simulink model "GFMUPS100k_CPP"  (R2024b)
settings: Solver=ode2  StartTime=0.0  StopTime=6  FixedStep=5e-7  RelTol=1e-3
model workspace (MAT data in the model file):
  amp = 0
  f1 = 1000
undefined symbols (not defined in the file or in its folder): DiscIntNeverNeededParam, L
libraries: spsIGBTDiodeLib x12, slpidlib x12, spsabctodq0Lib x10, spsSeriesRLCBranchLib x9, spsPLL3phLib x8, spsThreePhaseSeriesRLCBranchLib x8, spsDiodeLib x6, dspstat3 x5, spsVoltageMeasurementLib x4, spsThreePhaseVIMeasurementLib x4, spsPower3phInstantaneousLib x3, spsControlledCurrentSourceLib x3
(part 2 of 4)

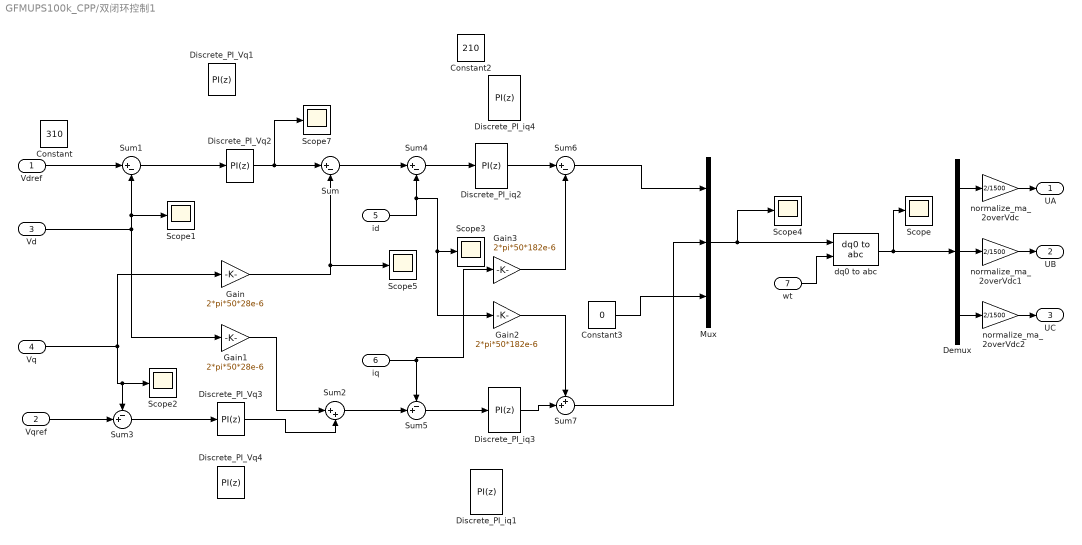
== system GFMUPS100k_CPP/双闭环控制1 ==
  Vdref : Inport
  Vqref : Inport  Port=2
  Vd : Inport  Port=3
  Vq : Inport  Port=4
  id : Inport  Port=5
  iq : Inport  Port=6
  wt : Inport  Port=7
  Constant : Constant  Value=310
  Constant2 : Constant  Value=210
  Constant3 : Constant  Value=0
  Demux : Demux  Outputs=3
  Discrete_PI_Vq1 : slpidlib/PID Controller  Controller=PI  Form=Parallel  TimeDomain=Discrete-time  UseExternalTs=off  SampleTime=5e-05  IntegratorMethod=Forward Euler  FilterMethod=Forward Euler  ControllerParametersSource=internal  P=0.16  I=500  UseKiTs=off  D=0  UseExternalDerivativeSource=off  N=100  UseFilter=on  TunerSelectOption=Transfer Function Based (PID Tuner App)  InitialConditionSource=internal  InitialConditionForIntegrator=0  InitialConditionForFilter=0  DifferentiatorICPrevScaledInput=0  ExternalReset=none  TrackingMode=off  Kt=1  LimitOutput=off  SatLimitsSource=internal  UpperSaturationLimit=inf  LowerSaturationLimit=-inf  LinearizeAsGain=off  AntiWindupMode=none  Kb=1  LimitIntegrator=off  UpperIntegratorSaturationLimit=inf  LowerIntegratorSaturationLimit=-inf  POutMin=[]  POutMax=[]  IOutMin=[]  IOutMax=[]  DOutMin=[]  DOutMax=[]  NOutMin=[]  NOutMax=[]  SumOutMin=[]  SumOutMax=[]  SaturationOutMin=[]  SaturationOutMax=[]  PParamMin=[]  PParamMax=[]  IParamMin=[]  IParamMax=[]  DParamMin=[]  DParamMax=[]  NParamMin=[]  NParamMax=[]  KbParamMin=[]  KbParamMax=[]  KtParamMin=[]  KtParamMax=[]  KbOutMin=[]  KbOutMax=[]  KtOutMin=[]  KtOutMax=[]  IntegratorOutMin=[]  IntegratorOutMax=[]  FilterOutMin=[]  FilterOutMax=[]  SumI1OutMin=[]  SumI1OutMax=[]  SumI2OutMin=[]  SumI2OutMax=[]  SumI3OutMin=[]  SumI3OutMax=[]  SumI4OutMin=[]  SumI4OutMax=[]  SumDOutMin=[]  SumDOutMax=[]  DifferentiatorOutMin=[]  DifferentiatorOutMax=[]  FilterDiffOutCoefMin=[]  FilterDiffOutCoefMax=[]  ReciprocalOutMin=[]  ReciprocalOutMax=[]  SumDenOutMin=[]  SumDenOutMax=[]  SumNumOutMin=[]  SumNumOutMax=[]  DivideOutMin=[]  DivideOutMax=[]  UdiffTsProdOutMin=[]  UdiffTsProdOutMax=[]  NTsProdOutMin=[]  NTsProdOutMax=[]  UintegralTsProdOutMin=[]  UintegralTsProdOutMax=[]  UngainTsProdOutMin=[]  UngainTsProdOutMax=[]  ClampingZeroOutDataTypeStr=Inherit: Inherit via back propagation  ClampingZeroOutMin=[]  ClampingZeroOutMax=[]  FilterDenConstantOutDataTypeStr=Inherit: Inherit via back propagation  FilterDenConstantOutMin=[]  FilterDenConstantOutMax=[]  PCopyOutDataTypeStr=Inherit: Inherit via back propagation  PCopyOutMin=[]  PCopyOutMax=[]  NCopyOutDataTypeStr=Inherit: Inherit via back propagation  NCopyOutMin=[]  NCopyOutMax=[]  IntegratorContinuousStateAttributes=''  IntegratorStateMustResolveToSignalObject=off  IntegratorRTWStateStorageClass=Auto  FilterContinuousStateAttributes=''  FilterStateMustResolveToSignalObject=off  FilterRTWStateStorageClass=Auto  ParallelPVariant=InternalParameters  IdealPVariant=Disabled  IVariant=InternalParameters  DVariant=Disabled  IntegratorVariant=Discrete  SatVariant=Disabled  AWVariant=Passthrough  PCopyVariant=Disabled  TRVariant=Disabled  FdbkBlocksVariant=Forward  IdealPFdbkVariant=Disabled  SatFdbkVariant=Disabled  DerivativeFilterVariant=Disabled  NVariant=Disabled  NCopyVariant=Disabled_SignalSpec  FilterICVariant=Disabled  IntegratorICVariant=InternalICs  ExternalResetVariant=Disabled  TRSumVariant=Passthrough  SumFdbkVariant=Disabled  SumVariant=Sum_PI  TsampFilterVariant=InternalTs  TsampNgainVariant=Passthrough  TsampIntegralVariant=Disabled_SignalSpec  ExternalSaturationOutDataTypeStr=Inherit: Same as second input  DerivativeSourceVariant=Disabled  PreIntVariant=InternalPreInt
  Discrete_PI_Vq2 : slpidlib/PID Controller  Controller=PI  Form=Parallel  TimeDomain=Discrete-time  UseExternalTs=off  SampleTime=5e-05  IntegratorMethod=Forward Euler  FilterMethod=Forward Euler  ControllerParametersSource=internal  P=0.16  I=250  UseKiTs=off  D=0  UseExternalDerivativeSource=off  N=100  UseFilter=on  TunerSelectOption=Transfer Function Based (PID Tuner App)  InitialConditionSource=internal  InitialConditionForIntegrator=0  InitialConditionForFilter=0  DifferentiatorICPrevScaledInput=0  ExternalReset=none  TrackingMode=off  Kt=1  LimitOutput=off  SatLimitsSource=internal  UpperSaturationLimit=inf  LowerSaturationLimit=-inf  LinearizeAsGain=off  AntiWindupMode=none  Kb=1  LimitIntegrator=off  UpperIntegratorSaturationLimit=inf  LowerIntegratorSaturationLimit=-inf  POutMin=[]  POutMax=[]  IOutMin=[]  IOutMax=[]  DOutMin=[]  DOutMax=[]  NOutMin=[]  NOutMax=[]  SumOutMin=[]  SumOutMax=[]  SaturationOutMin=[]  SaturationOutMax=[]  PParamMin=[]  PParamMax=[]  IParamMin=[]  IParamMax=[]  DParamMin=[]  DParamMax=[]  NParamMin=[]  NParamMax=[]  KbParamMin=[]  KbParamMax=[]  KtParamMin=[]  KtParamMax=[]  KbOutMin=[]  KbOutMax=[]  KtOutMin=[]  KtOutMax=[]  IntegratorOutMin=[]  IntegratorOutMax=[]  FilterOutMin=[]  FilterOutMax=[]  SumI1OutMin=[]  SumI1OutMax=[]  SumI2OutMin=[]  SumI2OutMax=[]  SumI3OutMin=[]  SumI3OutMax=[]  SumI4OutMin=[]  SumI4OutMax=[]  SumDOutMin=[]  SumDOutMax=[]  DifferentiatorOutMin=[]  DifferentiatorOutMax=[]  FilterDiffOutCoefMin=[]  FilterDiffOutCoefMax=[]  ReciprocalOutMin=[]  ReciprocalOutMax=[]  SumDenOutMin=[]  SumDenOutMax=[]  SumNumOutMin=[]  SumNumOutMax=[]  DivideOutMin=[]  DivideOutMax=[]  UdiffTsProdOutMin=[]  UdiffTsProdOutMax=[]  NTsProdOutMin=[]  NTsProdOutMax=[]  UintegralTsProdOutMin=[]  UintegralTsProdOutMax=[]  UngainTsProdOutMin=[]  UngainTsProdOutMax=[]  ClampingZeroOutDataTypeStr=Inherit: Inherit via back propagation  ClampingZeroOutMin=[]  ClampingZeroOutMax=[]  FilterDenConstantOutDataTypeStr=Inherit: Inherit via back propagation  FilterDenConstantOutMin=[]  FilterDenConstantOutMax=[]  PCopyOutDataTypeStr=Inherit: Inherit via back propagation  PCopyOutMin=[]  PCopyOutMax=[]  NCopyOutDataTypeStr=Inherit: Inherit via back propagation  NCopyOutMin=[]  NCopyOutMax=[]  IntegratorContinuousStateAttributes=''  IntegratorStateMustResolveToSignalObject=off  IntegratorRTWStateStorageClass=Auto  FilterContinuousStateAttributes=''  FilterStateMustResolveToSignalObject=off  FilterRTWStateStorageClass=Auto  ParallelPVariant=InternalParameters  IdealPVariant=Disabled  IVariant=InternalParameters  DVariant=Disabled  IntegratorVariant=Discrete  SatVariant=Disabled  AWVariant=Passthrough  PCopyVariant=Disabled  TRVariant=Disabled  FdbkBlocksVariant=Forward  IdealPFdbkVariant=Disabled  SatFdbkVariant=Disabled  DerivativeFilterVariant=Disabled  NVariant=Disabled  NCopyVariant=Disabled_SignalSpec  FilterICVariant=Disabled  IntegratorICVariant=InternalICs  ExternalResetVariant=Disabled  TRSumVariant=Passthrough  SumFdbkVariant=Disabled  SumVariant=Sum_PI  TsampFilterVariant=InternalTs  TsampNgainVariant=Passthrough  TsampIntegralVariant=Disabled_SignalSpec  ExternalSaturationOutDataTypeStr=Inherit: Same as second input  DerivativeSourceVariant=Disabled  PreIntVariant=InternalPreInt
  Discrete_PI_Vq3 : slpidlib/PID Controller  Controller=PI  Form=Parallel  TimeDomain=Discrete-time  UseExternalTs=off  SampleTime=5e-05  IntegratorMethod=Forward Euler  FilterMethod=Forward Euler  ControllerParametersSource=internal  P=0.16  I=250  UseKiTs=off  D=0  UseExternalDerivativeSource=off  N=100  UseFilter=on  TunerSelectOption=Transfer Function Based (PID Tuner App)  InitialConditionSource=internal  InitialConditionForIntegrator=0  InitialConditionForFilter=0  DifferentiatorICPrevScaledInput=0  ExternalReset=none  TrackingMode=off  Kt=1  LimitOutput=off  SatLimitsSource=internal  UpperSaturationLimit=inf  LowerSaturationLimit=-inf  LinearizeAsGain=off  AntiWindupMode=none  Kb=1  LimitIntegrator=off  UpperIntegratorSaturationLimit=inf  LowerIntegratorSaturationLimit=-inf  POutMin=[]  POutMax=[]  IOutMin=[]  IOutMax=[]  DOutMin=[]  DOutMax=[]  NOutMin=[]  NOutMax=[]  SumOutMin=[]  SumOutMax=[]  SaturationOutMin=[]  SaturationOutMax=[]  PParamMin=[]  PParamMax=[]  IParamMin=[]  IParamMax=[]  DParamMin=[]  DParamMax=[]  NParamMin=[]  NParamMax=[]  KbParamMin=[]  KbParamMax=[]  KtParamMin=[]  KtParamMax=[]  KbOutMin=[]  KbOutMax=[]  KtOutMin=[]  KtOutMax=[]  IntegratorOutMin=[]  IntegratorOutMax=[]  FilterOutMin=[]  FilterOutMax=[]  SumI1OutMin=[]  SumI1OutMax=[]  SumI2OutMin=[]  SumI2OutMax=[]  SumI3OutMin=[]  SumI3OutMax=[]  SumI4OutMin=[]  SumI4OutMax=[]  SumDOutMin=[]  SumDOutMax=[]  DifferentiatorOutMin=[]  DifferentiatorOutMax=[]  FilterDiffOutCoefMin=[]  FilterDiffOutCoefMax=[]  ReciprocalOutMin=[]  ReciprocalOutMax=[]  SumDenOutMin=[]  SumDenOutMax=[]  SumNumOutMin=[]  SumNumOutMax=[]  DivideOutMin=[]  DivideOutMax=[]  UdiffTsProdOutMin=[]  UdiffTsProdOutMax=[]  NTsProdOutMin=[]  NTsProdOutMax=[]  UintegralTsProdOutMin=[]  UintegralTsProdOutMax=[]  UngainTsProdOutMin=[]  UngainTsProdOutMax=[]  ClampingZeroOutDataTypeStr=Inherit: Inherit via back propagation  ClampingZeroOutMin=[]  ClampingZeroOutMax=[]  FilterDenConstantOutDataTypeStr=Inherit: Inherit via back propagation  FilterDenConstantOutMin=[]  FilterDenConstantOutMax=[]  PCopyOutDataTypeStr=Inherit: Inherit via back propagation  PCopyOutMin=[]  PCopyOutMax=[]  NCopyOutDataTypeStr=Inherit: Inherit via back propagation  NCopyOutMin=[]  NCopyOutMax=[]  IntegratorContinuousStateAttributes=''  IntegratorStateMustResolveToSignalObject=off  IntegratorRTWStateStorageClass=Auto  FilterContinuousStateAttributes=''  FilterStateMustResolveToSignalObject=off  FilterRTWStateStorageClass=Auto  ParallelPVariant=InternalParameters  IdealPVariant=Disabled  IVariant=InternalParameters  DVariant=Disabled  IntegratorVariant=Discrete  SatVariant=Disabled  AWVariant=Passthrough  PCopyVariant=Disabled  TRVariant=Disabled  FdbkBlocksVariant=Forward  IdealPFdbkVariant=Disabled  SatFdbkVariant=Disabled  DerivativeFilterVariant=Disabled  NVariant=Disabled  NCopyVariant=Disabled_SignalSpec  FilterICVariant=Disabled  IntegratorICVariant=InternalICs  ExternalResetVariant=Disabled  TRSumVariant=Passthrough  SumFdbkVariant=Disabled  SumVariant=Sum_PI  TsampFilterVariant=InternalTs  TsampNgainVariant=Passthrough  TsampIntegralVariant=Disabled_SignalSpec  ExternalSaturationOutDataTypeStr=Inherit: Same as second input  DerivativeSourceVariant=Disabled  PreIntVariant=InternalPreInt
  Discrete_PI_Vq4 : slpidlib/PID Controller  Controller=PI  Form=Parallel  TimeDomain=Discrete-time  UseExternalTs=off  SampleTime=5e-05  IntegratorMethod=Forward Euler  FilterMethod=Forward Euler  ControllerParametersSource=internal  P=0.16  I=500  UseKiTs=off  D=0  UseExternalDerivativeSource=off  N=100  UseFilter=on  TunerSelectOption=Transfer Function Based (PID Tuner App)  InitialConditionSource=internal  InitialConditionForIntegrator=0  InitialConditionForFilter=0  DifferentiatorICPrevScaledInput=0  ExternalReset=none  TrackingMode=off  Kt=1  LimitOutput=off  SatLimitsSource=internal  UpperSaturationLimit=inf  LowerSaturationLimit=-inf  LinearizeAsGain=off  AntiWindupMode=none  Kb=1  LimitIntegrator=off  UpperIntegratorSaturationLimit=inf  LowerIntegratorSaturationLimit=-inf  POutMin=[]  POutMax=[]  IOutMin=[]  IOutMax=[]  DOutMin=[]  DOutMax=[]  NOutMin=[]  NOutMax=[]  SumOutMin=[]  SumOutMax=[]  SaturationOutMin=[]  SaturationOutMax=[]  PParamMin=[]  PParamMax=[]  IParamMin=[]  IParamMax=[]  DParamMin=[]  DParamMax=[]  NParamMin=[]  NParamMax=[]  KbParamMin=[]  KbParamMax=[]  KtParamMin=[]  KtParamMax=[]  KbOutMin=[]  KbOutMax=[]  KtOutMin=[]  KtOutMax=[]  IntegratorOutMin=[]  IntegratorOutMax=[]  FilterOutMin=[]  FilterOutMax=[]  SumI1OutMin=[]  SumI1OutMax=[]  SumI2OutMin=[]  SumI2OutMax=[]  SumI3OutMin=[]  SumI3OutMax=[]  SumI4OutMin=[]  SumI4OutMax=[]  SumDOutMin=[]  SumDOutMax=[]  DifferentiatorOutMin=[]  DifferentiatorOutMax=[]  FilterDiffOutCoefMin=[]  FilterDiffOutCoefMax=[]  ReciprocalOutMin=[]  ReciprocalOutMax=[]  SumDenOutMin=[]  SumDenOutMax=[]  SumNumOutMin=[]  SumNumOutMax=[]  DivideOutMin=[]  DivideOutMax=[]  UdiffTsProdOutMin=[]  UdiffTsProdOutMax=[]  NTsProdOutMin=[]  NTsProdOutMax=[]  UintegralTsProdOutMin=[]  UintegralTsProdOutMax=[]  UngainTsProdOutMin=[]  UngainTsProdOutMax=[]  ClampingZeroOutDataTypeStr=Inherit: Inherit via back propagation  ClampingZeroOutMin=[]  ClampingZeroOutMax=[]  FilterDenConstantOutDataTypeStr=Inherit: Inherit via back propagation  FilterDenConstantOutMin=[]  FilterDenConstantOutMax=[]  PCopyOutDataTypeStr=Inherit: Inherit via back propagation  PCopyOutMin=[]  PCopyOutMax=[]  NCopyOutDataTypeStr=Inherit: Inherit via back propagation  NCopyOutMin=[]  NCopyOutMax=[]  IntegratorContinuousStateAttributes=''  IntegratorStateMustResolveToSignalObject=off  IntegratorRTWStateStorageClass=Auto  FilterContinuousStateAttributes=''  FilterStateMustResolveToSignalObject=off  FilterRTWStateStorageClass=Auto  ParallelPVariant=InternalParameters  IdealPVariant=Disabled  IVariant=InternalParameters  DVariant=Disabled  IntegratorVariant=Discrete  SatVariant=Disabled  AWVariant=Passthrough  PCopyVariant=Disabled  TRVariant=Disabled  FdbkBlocksVariant=Forward  IdealPFdbkVariant=Disabled  SatFdbkVariant=Disabled  DerivativeFilterVariant=Disabled  NVariant=Disabled  NCopyVariant=Disabled_SignalSpec  FilterICVariant=Disabled  IntegratorICVariant=InternalICs  ExternalResetVariant=Disabled  TRSumVariant=Passthrough  SumFdbkVariant=Disabled  SumVariant=Sum_PI  TsampFilterVariant=InternalTs  TsampNgainVariant=Passthrough  TsampIntegralVariant=Disabled_SignalSpec  ExternalSaturationOutDataTypeStr=Inherit: Same as second input  DerivativeSourceVariant=Disabled  PreIntVariant=InternalPreInt
  Discrete_PI_iq1 : slpidlib/PID Controller  Controller=PI  Form=Parallel  TimeDomain=Discrete-time  UseExternalTs=off  SampleTime=5e-05  IntegratorMethod=Forward Euler  FilterMethod=Forward Euler  ControllerParametersSource=internal  P=0.15  I=526*2  UseKiTs=off  D=0  UseExternalDerivativeSource=off  N=100  UseFilter=on  TunerSelectOption=Transfer Function Based (PID Tuner App)  InitialConditionSource=internal  InitialConditionForIntegrator=0  InitialConditionForFilter=0  DifferentiatorICPrevScaledInput=0  ExternalReset=none  TrackingMode=off  Kt=1  LimitOutput=off  SatLimitsSource=internal  UpperSaturationLimit=inf  LowerSaturationLimit=-inf  LinearizeAsGain=off  AntiWindupMode=none  Kb=1  LimitIntegrator=off  UpperIntegratorSaturationLimit=inf  LowerIntegratorSaturationLimit=-inf  POutMin=[]  POutMax=[]  IOutMin=[]  IOutMax=[]  DOutMin=[]  DOutMax=[]  NOutMin=[]  NOutMax=[]  SumOutMin=[]  SumOutMax=[]  SaturationOutMin=[]  SaturationOutMax=[]  PParamMin=[]  PParamMax=[]  IParamMin=[]  IParamMax=[]  DParamMin=[]  DParamMax=[]  NParamMin=[]  NParamMax=[]  KbParamMin=[]  KbParamMax=[]  KtParamMin=[]  KtParamMax=[]  KbOutMin=[]  KbOutMax=[]  KtOutMin=[]  KtOutMax=[]  IntegratorOutMin=[]  IntegratorOutMax=[]  FilterOutMin=[]  FilterOutMax=[]  SumI1OutMin=[]  SumI1OutMax=[]  SumI2OutMin=[]  SumI2OutMax=[]  SumI3OutMin=[]  SumI3OutMax=[]  SumI4OutMin=[]  SumI4OutMax=[]  SumDOutMin=[]  SumDOutMax=[]  DifferentiatorOutMin=[]  DifferentiatorOutMax=[]  FilterDiffOutCoefMin=[]  FilterDiffOutCoefMax=[]  ReciprocalOutMin=[]  ReciprocalOutMax=[]  SumDenOutMin=[]  SumDenOutMax=[]  SumNumOutMin=[]  SumNumOutMax=[]  DivideOutMin=[]  DivideOutMax=[]  UdiffTsProdOutMin=[]  UdiffTsProdOutMax=[]  NTsProdOutMin=[]  NTsProdOutMax=[]  UintegralTsProdOutMin=[]  UintegralTsProdOutMax=[]  UngainTsProdOutMin=[]  UngainTsProdOutMax=[]  ClampingZeroOutDataTypeStr=Inherit: Inherit via back propagation  ClampingZeroOutMin=[]  ClampingZeroOutMax=[]  FilterDenConstantOutDataTypeStr=Inherit: Inherit via back propagation  FilterDenConstantOutMin=[]  FilterDenConstantOutMax=[]  PCopyOutDataTypeStr=Inherit: Inherit via back propagation  PCopyOutMin=[]  PCopyOutMax=[]  NCopyOutDataTypeStr=Inherit: Inherit via back propagation  NCopyOutMin=[]  NCopyOutMax=[]  IntegratorContinuousStateAttributes=''  IntegratorStateMustResolveToSignalObject=off  IntegratorRTWStateStorageClass=Auto  FilterContinuousStateAttributes=''  FilterStateMustResolveToSignalObject=off  FilterRTWStateStorageClass=Auto  ParallelPVariant=InternalParameters  IdealPVariant=Disabled  IVariant=InternalParameters  DVariant=Disabled  IntegratorVariant=Discrete  SatVariant=Disabled  AWVariant=Passthrough  PCopyVariant=Disabled  TRVariant=Disabled  FdbkBlocksVariant=Forward  IdealPFdbkVariant=Disabled  SatFdbkVariant=Disabled  DerivativeFilterVariant=Disabled  NVariant=Disabled  NCopyVariant=Disabled_SignalSpec  FilterICVariant=Disabled  IntegratorICVariant=InternalICs  ExternalResetVariant=Disabled  TRSumVariant=Passthrough  SumFdbkVariant=Disabled  SumVariant=Sum_PI  TsampFilterVariant=InternalTs  TsampNgainVariant=Passthrough  TsampIntegralVariant=Disabled_SignalSpec  ExternalSaturationOutDataTypeStr=Inherit: Same as second input  DerivativeSourceVariant=Disabled  PreIntVariant=InternalPreInt
  Discrete_PI_iq2 : slpidlib/PID Controller  Controller=PI  Form=Parallel  TimeDomain=Discrete-time  UseExternalTs=off  SampleTime=5e-05  IntegratorMethod=Forward Euler  FilterMethod=Forward Euler  ControllerParametersSource=internal  P=1.2  I=526*2  UseKiTs=off  D=0  UseExternalDerivativeSource=off  N=100  UseFilter=on  TunerSelectOption=Transfer Function Based (PID Tuner App)  InitialConditionSource=internal  InitialConditionForIntegrator=0  InitialConditionForFilter=0  DifferentiatorICPrevScaledInput=0  ExternalReset=none  TrackingMode=off  Kt=1  LimitOutput=off  SatLimitsSource=internal  UpperSaturationLimit=inf  LowerSaturationLimit=-inf  LinearizeAsGain=off  AntiWindupMode=none  Kb=1  LimitIntegrator=off  UpperIntegratorSaturationLimit=inf  LowerIntegratorSaturationLimit=-inf  POutMin=[]  POutMax=[]  IOutMin=[]  IOutMax=[]  DOutMin=[]  DOutMax=[]  NOutMin=[]  NOutMax=[]  SumOutMin=[]  SumOutMax=[]  SaturationOutMin=[]  SaturationOutMax=[]  PParamMin=[]  PParamMax=[]  IParamMin=[]  IParamMax=[]  DParamMin=[]  DParamMax=[]  NParamMin=[]  NParamMax=[]  KbParamMin=[]  KbParamMax=[]  KtParamMin=[]  KtParamMax=[]  KbOutMin=[]  KbOutMax=[]  KtOutMin=[]  KtOutMax=[]  IntegratorOutMin=[]  IntegratorOutMax=[]  FilterOutMin=[]  FilterOutMax=[]  SumI1OutMin=[]  SumI1OutMax=[]  SumI2OutMin=[]  SumI2OutMax=[]  SumI3OutMin=[]  SumI3OutMax=[]  SumI4OutMin=[]  SumI4OutMax=[]  SumDOutMin=[]  SumDOutMax=[]  DifferentiatorOutMin=[]  DifferentiatorOutMax=[]  FilterDiffOutCoefMin=[]  FilterDiffOutCoefMax=[]  ReciprocalOutMin=[]  ReciprocalOutMax=[]  SumDenOutMin=[]  SumDenOutMax=[]  SumNumOutMin=[]  SumNumOutMax=[]  DivideOutMin=[]  DivideOutMax=[]  UdiffTsProdOutMin=[]  UdiffTsProdOutMax=[]  NTsProdOutMin=[]  NTsProdOutMax=[]  UintegralTsProdOutMin=[]  UintegralTsProdOutMax=[]  UngainTsProdOutMin=[]  UngainTsProdOutMax=[]  ClampingZeroOutDataTypeStr=Inherit: Inherit via back propagation  ClampingZeroOutMin=[]  ClampingZeroOutMax=[]  FilterDenConstantOutDataTypeStr=Inherit: Inherit via back propagation  FilterDenConstantOutMin=[]  FilterDenConstantOutMax=[]  PCopyOutDataTypeStr=Inherit: Inherit via back propagation  PCopyOutMin=[]  PCopyOutMax=[]  NCopyOutDataTypeStr=Inherit: Inherit via back propagation  NCopyOutMin=[]  NCopyOutMax=[]  IntegratorContinuousStateAttributes=''  IntegratorStateMustResolveToSignalObject=off  IntegratorRTWStateStorageClass=Auto  FilterContinuousStateAttributes=''  FilterStateMustResolveToSignalObject=off  FilterRTWStateStorageClass=Auto  ParallelPVariant=InternalParameters  IdealPVariant=Disabled  IVariant=InternalParameters  DVariant=Disabled  IntegratorVariant=Discrete  SatVariant=Disabled  AWVariant=Passthrough  PCopyVariant=Disabled  TRVariant=Disabled  FdbkBlocksVariant=Forward  IdealPFdbkVariant=Disabled  SatFdbkVariant=Disabled  DerivativeFilterVariant=Disabled  NVariant=Disabled  NCopyVariant=Disabled_SignalSpec  FilterICVariant=Disabled  IntegratorICVariant=InternalICs  ExternalResetVariant=Disabled  TRSumVariant=Passthrough  SumFdbkVariant=Disabled  SumVariant=Sum_PI  TsampFilterVariant=InternalTs  TsampNgainVariant=Passthrough  TsampIntegralVariant=Disabled_SignalSpec  ExternalSaturationOutDataTypeStr=Inherit: Same as second input  DerivativeSourceVariant=Disabled  PreIntVariant=InternalPreInt
  Discrete_PI_iq3 : slpidlib/PID Controller  Controller=PI  Form=Parallel  TimeDomain=Discrete-time  UseExternalTs=off  SampleTime=5e-05  IntegratorMethod=Forward Euler  FilterMethod=Forward Euler  ControllerParametersSource=internal  P=1.2  I=526*2  UseKiTs=off  D=0  UseExternalDerivativeSource=off  N=100  UseFilter=on  TunerSelectOption=Transfer Function Based (PID Tuner App)  InitialConditionSource=internal  InitialConditionForIntegrator=0  InitialConditionForFilter=0  DifferentiatorICPrevScaledInput=0  ExternalReset=none  TrackingMode=off  Kt=1  LimitOutput=off  SatLimitsSource=internal  UpperSaturationLimit=inf  LowerSaturationLimit=-inf  LinearizeAsGain=off  AntiWindupMode=none  Kb=1  LimitIntegrator=off  UpperIntegratorSaturationLimit=inf  LowerIntegratorSaturationLimit=-inf  POutMin=[]  POutMax=[]  IOutMin=[]  IOutMax=[]  DOutMin=[]  DOutMax=[]  NOutMin=[]  NOutMax=[]  SumOutMin=[]  SumOutMax=[]  SaturationOutMin=[]  SaturationOutMax=[]  PParamMin=[]  PParamMax=[]  IParamMin=[]  IParamMax=[]  DParamMin=[]  DParamMax=[]  NParamMin=[]  NParamMax=[]  KbParamMin=[]  KbParamMax=[]  KtParamMin=[]  KtParamMax=[]  KbOutMin=[]  KbOutMax=[]  KtOutMin=[]  KtOutMax=[]  IntegratorOutMin=[]  IntegratorOutMax=[]  FilterOutMin=[]  FilterOutMax=[]  SumI1OutMin=[]  SumI1OutMax=[]  SumI2OutMin=[]  SumI2OutMax=[]  SumI3OutMin=[]  SumI3OutMax=[]  SumI4OutMin=[]  SumI4OutMax=[]  SumDOutMin=[]  SumDOutMax=[]  DifferentiatorOutMin=[]  DifferentiatorOutMax=[]  FilterDiffOutCoefMin=[]  FilterDiffOutCoefMax=[]  ReciprocalOutMin=[]  ReciprocalOutMax=[]  SumDenOutMin=[]  SumDenOutMax=[]  SumNumOutMin=[]  SumNumOutMax=[]  DivideOutMin=[]  DivideOutMax=[]  UdiffTsProdOutMin=[]  UdiffTsProdOutMax=[]  NTsProdOutMin=[]  NTsProdOutMax=[]  UintegralTsProdOutMin=[]  UintegralTsProdOutMax=[]  UngainTsProdOutMin=[]  UngainTsProdOutMax=[]  ClampingZeroOutDataTypeStr=Inherit: Inherit via back propagation  ClampingZeroOutMin=[]  ClampingZeroOutMax=[]  FilterDenConstantOutDataTypeStr=Inherit: Inherit via back propagation  FilterDenConstantOutMin=[]  FilterDenConstantOutMax=[]  PCopyOutDataTypeStr=Inherit: Inherit via back propagation  PCopyOutMin=[]  PCopyOutMax=[]  NCopyOutDataTypeStr=Inherit: Inherit via back propagation  NCopyOutMin=[]  NCopyOutMax=[]  IntegratorContinuousStateAttributes=''  IntegratorStateMustResolveToSignalObject=off  IntegratorRTWStateStorageClass=Auto  FilterContinuousStateAttributes=''  FilterStateMustResolveToSignalObject=off  FilterRTWStateStorageClass=Auto  ParallelPVariant=InternalParameters  IdealPVariant=Disabled  IVariant=InternalParameters  DVariant=Disabled  IntegratorVariant=Discrete  SatVariant=Disabled  AWVariant=Passthrough  PCopyVariant=Disabled  TRVariant=Disabled  FdbkBlocksVariant=Forward  IdealPFdbkVariant=Disabled  SatFdbkVariant=Disabled  DerivativeFilterVariant=Disabled  NVariant=Disabled  NCopyVariant=Disabled_SignalSpec  FilterICVariant=Disabled  IntegratorICVariant=InternalICs  ExternalResetVariant=Disabled  TRSumVariant=Passthrough  SumFdbkVariant=Disabled  SumVariant=Sum_PI  TsampFilterVariant=InternalTs  TsampNgainVariant=Passthrough  TsampIntegralVariant=Disabled_SignalSpec  ExternalSaturationOutDataTypeStr=Inherit: Same as second input  DerivativeSourceVariant=Disabled  PreIntVariant=InternalPreInt
  Discrete_PI_iq4 : slpidlib/PID Controller  Controller=PI  Form=Parallel  TimeDomain=Discrete-time  UseExternalTs=off  SampleTime=5e-05  IntegratorMethod=Forward Euler  FilterMethod=Forward Euler  ControllerParametersSource=internal  P=0.15  I=526*2  UseKiTs=off  D=0  UseExternalDerivativeSource=off  N=100  UseFilter=on  TunerSelectOption=Transfer Function Based (PID Tuner App)  InitialConditionSource=internal  InitialConditionForIntegrator=0  InitialConditionForFilter=0  DifferentiatorICPrevScaledInput=0  ExternalReset=none  TrackingMode=off  Kt=1  LimitOutput=off  SatLimitsSource=internal  UpperSaturationLimit=inf  LowerSaturationLimit=-inf  LinearizeAsGain=off  AntiWindupMode=none  Kb=1  LimitIntegrator=off  UpperIntegratorSaturationLimit=inf  LowerIntegratorSaturationLimit=-inf  POutMin=[]  POutMax=[]  IOutMin=[]  IOutMax=[]  DOutMin=[]  DOutMax=[]  NOutMin=[]  NOutMax=[]  SumOutMin=[]  SumOutMax=[]  SaturationOutMin=[]  SaturationOutMax=[]  PParamMin=[]  PParamMax=[]  IParamMin=[]  IParamMax=[]  DParamMin=[]  DParamMax=[]  NParamMin=[]  NParamMax=[]  KbParamMin=[]  KbParamMax=[]  KtParamMin=[]  KtParamMax=[]  KbOutMin=[]  KbOutMax=[]  KtOutMin=[]  KtOutMax=[]  IntegratorOutMin=[]  IntegratorOutMax=[]  FilterOutMin=[]  FilterOutMax=[]  SumI1OutMin=[]  SumI1OutMax=[]  SumI2OutMin=[]  SumI2OutMax=[]  SumI3OutMin=[]  SumI3OutMax=[]  SumI4OutMin=[]  SumI4OutMax=[]  SumDOutMin=[]  SumDOutMax=[]  DifferentiatorOutMin=[]  DifferentiatorOutMax=[]  FilterDiffOutCoefMin=[]  FilterDiffOutCoefMax=[]  ReciprocalOutMin=[]  ReciprocalOutMax=[]  SumDenOutMin=[]  SumDenOutMax=[]  SumNumOutMin=[]  SumNumOutMax=[]  DivideOutMin=[]  DivideOutMax=[]  UdiffTsProdOutMin=[]  UdiffTsProdOutMax=[]  NTsProdOutMin=[]  NTsProdOutMax=[]  UintegralTsProdOutMin=[]  UintegralTsProdOutMax=[]  UngainTsProdOutMin=[]  UngainTsProdOutMax=[]  ClampingZeroOutDataTypeStr=Inherit: Inherit via back propagation  ClampingZeroOutMin=[]  ClampingZeroOutMax=[]  FilterDenConstantOutDataTypeStr=Inherit: Inherit via back propagation  FilterDenConstantOutMin=[]  FilterDenConstantOutMax=[]  PCopyOutDataTypeStr=Inherit: Inherit via back propagation  PCopyOutMin=[]  PCopyOutMax=[]  NCopyOutDataTypeStr=Inherit: Inherit via back propagation  NCopyOutMin=[]  NCopyOutMax=[]  IntegratorContinuousStateAttributes=''  IntegratorStateMustResolveToSignalObject=off  IntegratorRTWStateStorageClass=Auto  FilterContinuousStateAttributes=''  FilterStateMustResolveToSignalObject=off  FilterRTWStateStorageClass=Auto  ParallelPVariant=InternalParameters  IdealPVariant=Disabled  IVariant=InternalParameters  DVariant=Disabled  IntegratorVariant=Discrete  SatVariant=Disabled  AWVariant=Passthrough  PCopyVariant=Disabled  TRVariant=Disabled  FdbkBlocksVariant=Forward  IdealPFdbkVariant=Disabled  SatFdbkVariant=Disabled  DerivativeFilterVariant=Disabled  NVariant=Disabled  NCopyVariant=Disabled_SignalSpec  FilterICVariant=Disabled  IntegratorICVariant=InternalICs  ExternalResetVariant=Disabled  TRSumVariant=Passthrough  SumFdbkVariant=Disabled  SumVariant=Sum_PI  TsampFilterVariant=InternalTs  TsampNgainVariant=Passthrough  TsampIntegralVariant=Disabled_SignalSpec  ExternalSaturationOutDataTypeStr=Inherit: Same as second input  DerivativeSourceVariant=Disabled  PreIntVariant=InternalPreInt
  Gain : Gain  Gain=2*pi*50*28e-6
  Gain1 : Gain  Gain=2*pi*50*28e-6
  Gain2 : Gain  Gain=2*pi*50*182e-6
  Gain3 : Gain  Gain=2*pi*50*182e-6
  Mux : Mux  Inputs=3
  Scope{,1..5,7} (7 alike) : Scope
  Sum{,1,4,6} (4 alike) : Sum  Inputs=|+-
  Sum2 : Sum  Inputs=|++
  Sum3 : Sum  Inputs=-+|
  Sum5 : Sum  Inputs=-+|
  Sum7 : Sum  Inputs=++|
  dq0 to abc : spsdq0toabcLib/dq0 to abc  Alignment=90 degrees behind phase A axis
  normalize_ma_2overVdc : Gain  Gain=2/1500
  normalize_ma_2overVdc1 : Gain  Gain=2/1500
  normalize_ma_2overVdc2 : Gain  Gain=2/1500
  UA : Outport
  UB : Outport  Port=2
  UC : Outport  Port=3
  wires:
  Sum/1 -> Sum4/1
  Constant3/1 -> Mux/3
  Sum2/1 -> Sum5/2
  Gain1/1 -> Sum2/1
  Mux/1 -> dq0 to abc/1, Scope4/1
  Vqref/1 -> Sum3/2
  Vdref/1 -> Sum1/1
  normalize_ma_2overVdc2/1 -> UC/1
  normalize_ma_2overVdc1/1 -> UB/1
  normalize_ma_2overVdc/1 -> UA/1
  Gain/1 -> Scope5/1, Sum/2
  Sum1/1 -> Discrete_PI_Vq2/1
  Vd/1 -> Gain1/1, Scope1/1, Sum1/2
  Vq/1 -> Gain/1, Sum3/1, Scope2/1
  wt/1 -> dq0 to abc/2
  iq/1 -> Sum5/1, Gain3/1
  Demux/2 -> normalize_ma_2overVdc1/1
  Discrete_PI_Vq2/1 -> Scope7/1, Sum/1
  Sum5/1 -> Discrete_PI_iq3/1
  dq0 to abc/1 -> Demux/1, Scope/1
  Discrete_PI_Vq3/1 -> Sum2/2
  Demux/1 -> normalize_ma_2overVdc/1
  Demux/3 -> normalize_ma_2overVdc2/1
  Sum4/1 -> Discrete_PI_iq2/1
  Sum3/1 -> Discrete_PI_Vq3/1
  id/1 -> Gain2/1, Scope3/1, Sum4/2
  Discrete_PI_iq2/1 -> Sum6/1
  Discrete_PI_iq3/1 -> Sum7/2
  Sum7/1 -> Mux/2
  Sum6/1 -> Mux/1
  Gain2/1 -> Sum7/1
  Gain3/1 -> Sum6/2

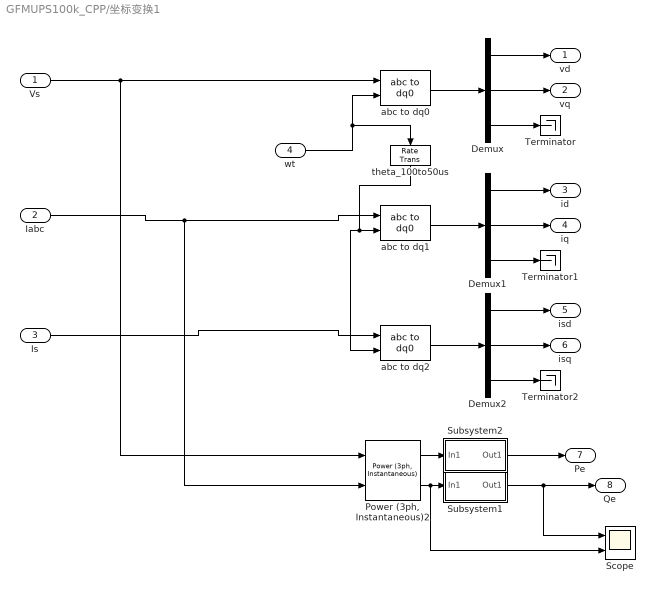
== system GFMUPS100k_CPP/坐标变换1 ==
  Vs : Inport
  Iabc : Inport  Port=2
  Is : Inport  Port=3
  wt : Inport  Port=4
  Demux : Demux  Outputs=3
  Demux1 : Demux  Outputs=3
  Demux2 : Demux  Outputs=3
  "Power (3ph, Instantaneous)2" : spsPower3phInstantaneousLib/Power (3ph, Instantaneous)
  Scope : Scope  NumInputPorts=2
  Subsystem1 : Subsystem
  Subsystem2 : Subsystem
  Terminator : Terminator
  Terminator1 : Terminator
  Terminator2 : Terminator
  abc to dq0 : spsabctodq0Lib/abc to dq0  Alignment=90 degrees behind phase A axis
  abc to dq1 : spsabctodq0Lib/abc to dq0  Alignment=90 degrees behind phase A axis
  abc to dq2 : spsabctodq0Lib/abc to dq0  Alignment=90 degrees behind phase A axis
  theta_100to50us : RateTransition  OutPortSampleTime=50e-6
  vd : Outport
  vq : Outport  Port=2
  id : Outport  Port=3
  iq : Outport  Port=4
  isd : Outport  Port=5
  isq : Outport  Port=6
  Pe : Outport  Port=7
  Qe : Outport  Port=8
  wires:
  Demux/3 -> Terminator/1
  Demux2/3 -> Terminator2/1
  wt/1 -> abc to dq0/2, theta_100to50us/1
  "Power (3ph, Instantaneous)2"/1 -> Subsystem2/1(In1)
  "Power (3ph, Instantaneous)2"/2 -> Scope/2, Subsystem1/1(In1)
  Demux/1 -> vd/1
  Demux1/1 -> id/1
  Demux2/1 -> isd/1
  abc to dq0/1 -> Demux/1
  Vs/1 -> abc to dq0/1, "Power (3ph, Instantaneous)2"/1
  Demux/2 -> vq/1
  Is/1 -> abc to dq2/1
  Demux2/2 -> isq/1
  abc to dq2/1 -> Demux2/1
  Iabc/1 -> abc to dq1/1, "Power (3ph, Instantaneous)2"/2
  abc to dq1/1 -> Demux1/1
  Demux1/3 -> Terminator1/1
  Demux1/2 -> iq/1
  theta_100to50us/1 -> abc to dq2/2, abc to dq1/2
  Subsystem2/1(Out1) -> Pe/1
  Subsystem1/1(Out1) -> Scope/1, Qe/1

== system GFMUPS100k_CPP/基于自适应虚拟电流 ==
  presignal : Inport
  Vs_abc : Inport  Port=2
  Vg_abc1 : Inport  Port=3
  Constant1 : Constant  Value=1.8
  Constant2 : Constant  Value=0.01
  Gain1 : Gain  Gain=314.16
  MATLAB Function : MATLAB Function  TreatAsAtomicUnit=on
  PLL (3ph) : spsPLL3phLib/PLL (3ph)  Fmin=45  Par_Init=[0, 60]  ParK=[180, 3200, 1]  TcD=1e-4  MaxRateChangeFreq=12  FilterCutOffFreq=25  Ts=0  AGC=on
  Scope2 : Scope  NumInputPorts=3
  Scope3 : Scope
  Terminator8 : Terminator
  d轴电压 : Subsystem
  todq : Subsystem
  标幺 : Subsystem
  自适应PI : Subsystem
  重构 : MATLAB Function  TreatAsAtomicUnit=on  SystemSampleTime=5e-05
  deta_U : Outport
  deta_w : Outport  Port=2
  wires:
  todq/2(Iq) -> 重构/2(Ivq), Scope2/2
  todq/3(Iv) -> 重构/3(Iv), Scope2/3
  todq/1(Id) -> Scope2/1, d轴电压/2(Ivd), 重构/1(Ivd)
  标幺/4(Vg_beta1) -> todq/5(psi_Vg_Beta)
  标幺/3(Vg_alpha1) -> todq/4(psi_Vg_Alpha)
  标幺/2(Vs_beta) -> todq/3(psi_VS_Beta)
  标幺/1(Vs_alpha) -> todq/2(psi_VS_Alpha)
  PLL (3ph)/2 -> todq/1(wt)
  PLL (3ph)/1 -> Terminator8/1
  Vg_abc1/1 -> 标幺/2(abc1)
  d轴电压/1("deta U ") -> deta_U/1
  Vs_abc/1 -> 标幺/1(abc), PLL (3ph)/1
  MATLAB Function/1(y) -> deta_w/1
  Gain1/1 -> Scope3/1, MATLAB Function/1(u)
  重构/1(Ivq_re) -> 自适应PI/1(Ivq_re)
  Constant1/1 -> 自适应PI/2(Kp_base)
  Constant2/1 -> 自适应PI/3(Ki_base)
  自适应PI/1(Out1) -> Gain1/1
  presignal/1 -> d轴电压/1(presignal), MATLAB Function/2(presignal)

== system GFMUPS100k_CPP/基于转dq的预同步控制1 ==
  Vg : Inport
  Vabc : Inport  Port=2
  presignal : Inport  Port=3
  电压预同步 : Subsystem
  相位预同步 : Subsystem
  c_theta : Outport
  d_U : Outport  Port=2
  wires:
  电压预同步/1(d_U) -> d_U/1
  Vg/1 -> 相位预同步/1(Vg), 电压预同步/1(Vg)
  presignal/1 -> 相位预同步/3(presignal), 电压预同步/3(presignal)
  Vabc/1 -> 电压预同步/2(Vabc), 相位预同步/2(Vabc)
  相位预同步/1(c_theta) -> c_theta/1

== system GFMUPS100k_CPP/幅值差计算 ==
  In1 : Inport
  In2 : Inport  Port=2
  RMS1 : dspstat3/RMS  run=off  directionMode=Each column  dimension=1  InputProcessing=Columns as channels (frame based)  reset_popup=None
  RMS2 : dspstat3/RMS  run=off  directionMode=Each column  dimension=1  InputProcessing=Columns as channels (frame based)  reset_popup=None
  Sum4 : Sum  Inputs=|+-
  Out1 : Outport
  wires:
  RMS2/1 -> Sum4/1
  RMS1/1 -> Sum4/2
  In1/1 -> RMS2/1
  In2/1 -> RMS1/1
  Sum4/1 -> Out1/1

== system GFMUPS100k_CPP/正序扰动 ==
  Controlled Current Source1 : spsControlledCurrentSourceLib/Controlled Current Source  Initialize=on  Source_Type=AC  Amplitude=0  Phase=0  Frequency=0  Measurements=None
  Controlled Current Source2 : spsControlledCurrentSourceLib/Controlled Current Source  Initialize=on  Source_Type=AC  Amplitude=0  Phase=0  Frequency=0  Measurements=None
  Controlled Current Source3 : spsControlledCurrentSourceLib/Controlled Current Source  Initialize=on  Source_Type=AC  Amplitude=0  Phase=0  Frequency=0  Measurements=None
  Sine Wave : Sin  SampleTime=0
  Connection Port : PMIOPort  Side=Right
  Connection Port1 : PMIOPort  Port=2  Side=Right
  Connection Port2 : PMIOPort  Port=3  Side=Right
  Connection Port3 : PMIOPort  Port=4  Side=Left
  Connection Port4 : PMIOPort  Port=5  Side=Left
  Connection Port5 : PMIOPort  Port=6  Side=Left
  wires:
  Sine Wave/1 -> Controlled Current Source3/1, Controlled Current Source2/1, Controlled Current Source1/1
  connections:
  Connection Port2/RConn1 -- Controlled Current Source3/LConn1
  Connection Port1/RConn1 -- Controlled Current Source2/LConn1
  Connection Port3/RConn1 -- Controlled Current Source1/RConn1
  Connection Port/RConn1 -- Controlled Current Source1/LConn1
  Connection Port4/RConn1 -- Controlled Current Source2/RConn1
  Connection Port5/RConn1 -- Controlled Current Source3/RConn1

== system GFMUPS100k_CPP/正序扰动1 ==
  Controlled Voltage Source1 : spsControlledVoltageSourceLib/Controlled Voltage Source  Initialize=on  Source_Type=AC  Amplitude=0  Phase=0  Frequency=0  Measurements=None
  Controlled Voltage Source2 : spsControlledVoltageSourceLib/Controlled Voltage Source  Initialize=on  Source_Type=AC  Amplitude=0  Phase=0  Frequency=0  Measurements=None
  Controlled Voltage Source3 : spsControlledVoltageSourceLib/Controlled Voltage Source  Initialize=on  Source_Type=AC  Amplitude=0  Phase=0  Frequency=0  Measurements=None
  Divide : Product  Inputs=**
  Divide1 : Product  Inputs=**
  Divide2 : Product  Inputs=**
  Sine Wave : Sin  Amplitude=amp  Frequency=2*pi*f1  SampleTime=0
  Sine Wave1 : Sin  Amplitude=amp  Frequency=2*pi*f1  Phase=-2*pi/3  SampleTime=0
  Sine Wave2 : Sin  Amplitude=amp  Frequency=2*pi*f1  Phase=2*pi/3  SampleTime=0
  Step : Step  Time=2  SampleTime=0
  a : PMIOPort  Side=Right
  b : PMIOPort  Port=2  Side=Right
  c : PMIOPort  Port=3  Side=Right
  A : PMIOPort  Port=4  Side=Left
  B : PMIOPort  Port=5  Side=Left
  C : PMIOPort  Port=6  Side=Left
  wires:
  Sine Wave/1 -> Divide/2
  Step/1 -> Divide2/1, Divide/1, Divide1/1
  Sine Wave1/1 -> Divide1/2
  Sine Wave2/1 -> Divide2/2
  Divide2/1 -> Controlled Voltage Source3/1
  Divide1/1 -> Controlled Voltage Source2/1
  Divide/1 -> Controlled Voltage Source1/1
  connections:
  Controlled Voltage Source3/RConn1 -- C/RConn1
  Controlled Voltage Source2/RConn1 -- B/RConn1
  Controlled Voltage Source1/LConn1 -- a/RConn1
  Controlled Voltage Source1/RConn1 -- A/RConn1
  Controlled Voltage Source2/LConn1 -- b/RConn1
  Controlled Voltage Source3/LConn1 -- c/RConn1

== system GFMUPS100k_CPP/相角差计算 ==
  abc : Inport
  abc1 : Inport  Port=2
  Derivative : Derivative
  Sin : Trigonometry
  Subsystem1 : Subsystem
  Subsystem2 : Subsystem
  dete_theta : Outport
  Out2 : Outport  Port=2
  Out3 : Outport  Port=3
  Out4 : Outport  Port=4
  wires:
  abc1/1 -> Subsystem1/2(abc1)
  Sin/1 -> Out3/1, Derivative/1
  Subsystem1/1(Out1) -> Sin/1, Out2/1, Subsystem2/1(In1)
  abc/1 -> Subsystem1/1(abc)
  Subsystem2/1(dete_theta) -> dete_theta/1
  Derivative/1 -> Out4/1

== system GFMUPS100k_CPP/频率差计算 ==
  In1 : Inport
  In2 : Inport  Port=2
  Add : Sum  Inputs=+-
  Out1 : Outport
  wires:
  Add/1 -> Out1/1
  In2/1 -> Add/2
  In1/1 -> Add/1

== system GFMUPS100k_CPP/A practical and fast sequence components detection scheme for three-phase unbalanced grid voltage.2021/Subsystem ==
  abc : Inport
  Demux : Demux  Outputs=3
  MATLAB Function1 : MATLAB Function  TreatAsAtomicUnit=on
  MATLAB Function2 : MATLAB Function  TreatAsAtomicUnit=on
  PLL (3ph) : spsPLL3phLib/PLL (3ph)  Fmin=45  Par_Init=[0, 60]  ParK=[180, 3200, 1]  TcD=1e-4  MaxRateChangeFreq=12  FilterCutOffFreq=25  Ts=0  AGC=on
  Terminator : Terminator
  Terminator1 : Terminator
  abc to dq0 : spsabctodq0Lib/abc to dq0  Alignment=90 degrees behind phase A axis
  ud_fliter : Outport
  uq_fliter : Outport  Port=2
  wires:
  PLL (3ph)/1 -> Terminator/1
  Demux/2 -> MATLAB Function2/1(u)
  abc/1 -> PLL (3ph)/1, abc to dq0/1
  Demux/3 -> Terminator1/1
  Demux/1 -> MATLAB Function1/1(u)
  abc to dq0/1 -> Demux/1
  PLL (3ph)/2 -> abc to dq0/2
  MATLAB Function1/1(y_out) -> ud_fliter/1
  MATLAB Function2/1(y_out) -> uq_fliter/1

== system GFMUPS100k_CPP/A practical and fast sequence components detection scheme for three-phase unbalanced grid voltage.2021/Subsystem1 ==
  abc : Inport
  In1 : Inport  Port=2
  Demux : Demux  Outputs=3
  Demux1 : Demux  Outputs=3
  Gain : Gain  Gain=-1
  MATLAB Function1 : MATLAB Function  TreatAsAtomicUnit=on
  MATLAB Function2 : MATLAB Function  TreatAsAtomicUnit=on
  Mux : Mux  Inputs=3
  PLL (3ph) : spsPLL3phLib/PLL (3ph)  Commented=on  Fmin=45  Par_Init=[0, 60]  ParK=[180, 3200, 1]  TcD=1e-4  MaxRateChangeFreq=12  FilterCutOffFreq=25  Ts=0  AGC=on
  Terminator : Terminator  Commented=on
  Terminator1 : Terminator
  abc to dq0 : spsabctodq0Lib/abc to dq0  Alignment=90 degrees behind phase A axis
  ud_fliter : Outport
  uq_fliter : Outport  Port=2
  wires:
  MATLAB Function2/1(y_out) -> uq_fliter/1
  MATLAB Function1/1(y_out) -> ud_fliter/1
  abc to dq0/1 -> Demux/1
  Demux/1 -> MATLAB Function1/1(u)
  Demux/3 -> Terminator1/1
  Demux/2 -> MATLAB Function2/1(u)
  Gain/1 -> abc to dq0/2
  PLL (3ph)/1 -> Terminator/1
  abc/1 -> Demux1/1
  Demux1/1 -> Mux/1
  In1/1 -> Gain/1
  Mux/1 -> abc to dq0/1
  Demux1/2 -> Mux/2
  Demux1/3 -> Mux/3

== system GFMUPS100k_CPP/A practical and fast sequence components detection scheme for three-phase unbalanced grid voltage.2021/Ubeta计算 ==
  In1 : Inport
  Constant1 : Constant  Value=20
  Constant10 : Constant  Value=1e-4
  Constant11 : Constant  Value=2*pi*50
  Constant2 : Constant  Value=20
  Constant3 : Constant  Value=20
  Constant6 : Constant  Value=1e-4
  Constant7 : Constant  Value=2*pi*50
  Constant8 : Constant  Value=1e-4
  Constant9 : Constant  Value=2*pi*50
  Demux4 : Demux  Outputs=3
  MATLAB Function10 : MATLAB Function  TreatAsAtomicUnit=on  SystemSampleTime=1e-4
  MATLAB Function11 : MATLAB Function  TreatAsAtomicUnit=on  SystemSampleTime=1e-4
  MATLAB Function9 : MATLAB Function  TreatAsAtomicUnit=on  SystemSampleTime=1e-4
  uA_beta : Outport
  uB_beta : Outport  Port=2
  uC_beta : Outport  Port=3
  wires:
  MATLAB Function11/1(u_beta) -> uC_beta/1
  In1/1 -> Demux4/1
  MATLAB Function9/1(u_beta) -> uA_beta/1
  MATLAB Function10/1(u_beta) -> uB_beta/1
  Demux4/1 -> MATLAB Function9/1(u_alpha)
  Constant7/1 -> MATLAB Function9/3(omega)
  Constant6/1 -> MATLAB Function9/2(Ts)
  Constant11/1 -> MATLAB Function11/3(omega)
  Demux4/3 -> MATLAB Function11/1(u_alpha)
  Constant8/1 -> MATLAB Function10/2(Ts)
  Constant9/1 -> MATLAB Function10/3(omega)
  Constant10/1 -> MATLAB Function11/2(Ts)
  Demux4/2 -> MATLAB Function10/1(u_alpha)
  Constant1/1 -> MATLAB Function9/4(N)
  Constant2/1 -> MATLAB Function10/4(N)
  Constant3/1 -> MATLAB Function11/4(N)

== system GFMUPS100k_CPP/A practical and fast sequence components detection scheme for three-phase unbalanced grid voltage.2021/标幺化1 ==
  In1 : Inport
  Demux3 : Demux  Outputs=3
  Gain1 : Gain  Gain=1/311
  Gain2 : Gain  Gain=1/311
  Gain3 : Gain  Gain=1/311
  Mux : Mux  Inputs=3
  U_alpha : Outport
  wires:
  Gain3/1 -> Mux/3
  Gain1/1 -> Mux/2
  In1/1 -> Demux3/1
  Gain2/1 -> Mux/1
  Demux3/3 -> Gain3/1
  Demux3/2 -> Gain1/1
  Mux/1 -> U_alpha/1
  Demux3/1 -> Gain2/1

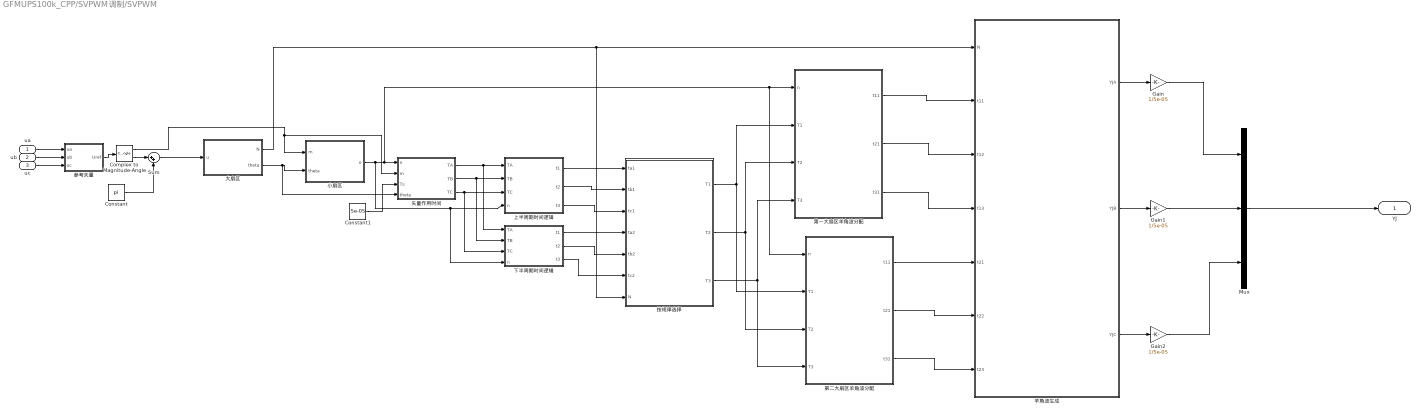
== system GFMUPS100k_CPP/SVPWM调制/SVPWM ==
  ua : Inport
  ub : Inport  Port=2
  uc : Inport  Port=3
  Complex to Magnitude-Angle : ComplexToMagnitudeAngle
  Constant : Constant  Value=pi
  Constant1 : Constant  Value=5e-05
  Gain : Gain  Gain=1/5e-05
  Gain1 : Gain  Gain=1/5e-05
  Gain2 : Gain  Gain=1/5e-05
  Mux : Mux  Inputs=3
  Sum : Sum  Inputs=|++
  上半周期时间逻辑 : MATLAB Function  TreatAsAtomicUnit=on
  下半周期时间逻辑 : MATLAB Function  TreatAsAtomicUnit=on
  参考矢量 : MATLAB Function  TreatAsAtomicUnit=on
  大扇区 : MATLAB Function  TreatAsAtomicUnit=on
  小扇区 : MATLAB Function  TreatAsAtomicUnit=on
  按规律选择 : MATLAB Function  TreatAsAtomicUnit=on
  矢量作用时间 : MATLAB Function  TreatAsAtomicUnit=on
  第一大扇区羊角波分配 : MATLAB Function  TreatAsAtomicUnit=on
  第二大扇区羊角波分配 : MATLAB Function  TreatAsAtomicUnit=on
  羊角波生成 : MATLAB Function  TreatAsAtomicUnit=on
  YJ : Outport
  wires:
  羊角波生成/2(YJB) -> Gain1/1
  矢量作用时间/1(TA) -> 下半周期时间逻辑/1(TA), 上半周期时间逻辑/1(TA)
  大扇区/1(N) -> 按规律选择/7(N), 羊角波生成/1(N)
  按规律选择/3(T3) -> 第一大扇区羊角波分配/4(T3), 第二大扇区羊角波分配/4(T3)
  Constant/1 -> Sum/2
  下半周期时间逻辑/1(t1) -> 按规律选择/4(ta2)
  大扇区/2(theta) -> 矢量作用时间/4(theta), 小扇区/2(theta)
  Gain2/1 -> Mux/3
  小扇区/1(n) -> 下半周期时间逻辑/4(n), 上半周期时间逻辑/4(n), 第二大扇区羊角波分配/1(n), 第一大扇区羊角波分配/1(n), 矢量作用时间/1(n)
  参考矢量/1(Uref) -> Complex to Magnitude-Angle/1
  uc/1 -> 参考矢量/3(uc)
  羊角波生成/3(YJC) -> Gain2/1
  羊角波生成/1(YJA) -> Gain/1
  Gain1/1 -> Mux/2
  Complex to Magnitude-Angle/1 -> 小扇区/1(m), 矢量作用时间/2(m)
  第二大扇区羊角波分配/2(t21) -> 羊角波生成/6(t22)
  按规律选择/2(T2) -> 第二大扇区羊角波分配/3(T2), 第一大扇区羊角波分配/3(T2)
  按规律选择/1(T1) -> 第二大扇区羊角波分配/2(T1), 第一大扇区羊角波分配/2(T1)
  矢量作用时间/2(TB) -> 下半周期时间逻辑/2(TB), 上半周期时间逻辑/2(TB)
  Gain/1 -> Mux/1
  Constant1/1 -> 矢量作用时间/3(Ts)
  第二大扇区羊角波分配/1(t11) -> 羊角波生成/5(t21)
  第一大扇区羊角波分配/3(t31) -> 羊角波生成/4(t13)
  ua/1 -> 参考矢量/1(ua)
  矢量作用时间/3(TC) -> 下半周期时间逻辑/3(TC), 上半周期时间逻辑/3(TC)
  第二大扇区羊角波分配/3(t31) -> 羊角波生成/7(t23)
  上半周期时间逻辑/2(t2) -> 按规律选择/2(tb1)
  上半周期时间逻辑/3(t3) -> 按规律选择/3(tc1)
  下半周期时间逻辑/2(t2) -> 按规律选择/5(tb2)
  Complex to Magnitude-Angle/2 -> Sum/1
  下半周期时间逻辑/3(t3) -> 按规律选择/6(tc2)
  上半周期时间逻辑/1(t1) -> 按规律选择/1(ta1)
  Mux/1 -> YJ/1
  Sum/1 -> 大扇区/1(u)
  第一大扇区羊角波分配/2(t21) -> 羊角波生成/3(t12)
  第一大扇区羊角波分配/1(t11) -> 羊角波生成/2(t11)
  ub/1 -> 参考矢量/2(ub)

== system GFMUPS100k_CPP/SVPWM调制/调制 ==
  YJ : Inport
  Constant : Constant
  Logical Operator : Logic  Operator=NOT  AllPortsSameDT=off  OutDataTypeStr=boolean
  Logical Operator1 : Logic  Operator=NOT  AllPortsSameDT=off  OutDataTypeStr=boolean
  Relational Operator : RelationalOperator  OutDataTypeStr=boolean  RndMeth=Simplest  InputSameDT=off
  Relational Operator1 : RelationalOperator  OutDataTypeStr=boolean  RndMeth=Simplest  InputSameDT=off
  Repeating Sequence : simulink/Sources/Repeating Sequence  rep_seq_t=[0 0.5*5e-5 5e-5]  rep_seq_y=[1 0 1]
  Saturation : Saturate  UpperLimit=1  LowerLimit=0
  Saturation1 : Saturate  UpperLimit=1  LowerLimit=0
  Scope : Scope  NumInputPorts=3
  Sum : Sum  Inputs=|++
  S1 : Outport
  S2 : Outport  Port=2
  S3 : Outport  Port=3
  S4 : Outport  Port=4
  wires:
  Sum/1 -> Saturation/1
  Saturation/1 -> Scope/1, Relational Operator/1
  YJ/1 -> Sum/2, Saturation1/1
  Saturation1/1 -> Scope/2, Relational Operator1/1
  Repeating Sequence/1 -> Relational Operator1/2, Scope/3, Relational Operator/2
  Relational Operator1/1 -> S1/1, Logical Operator1/1
  Logical Operator1/1 -> S3/1
  Relational Operator/1 -> S2/1, Logical Operator/1
  Logical Operator/1 -> S4/1
  Constant/1 -> Sum/1

== system GFMUPS100k_CPP/VSG_Control/Subsystem1 ==
  E : Inport
  Demux : Demux  Outputs=3
  Terminator : Terminator
  Ed : Outport
  Eq : Outport  Port=2
  wires:
  Demux/2 -> Eq/1
  E/1 -> Demux/1
  Demux/1 -> Ed/1
  Demux/3 -> Terminator/1

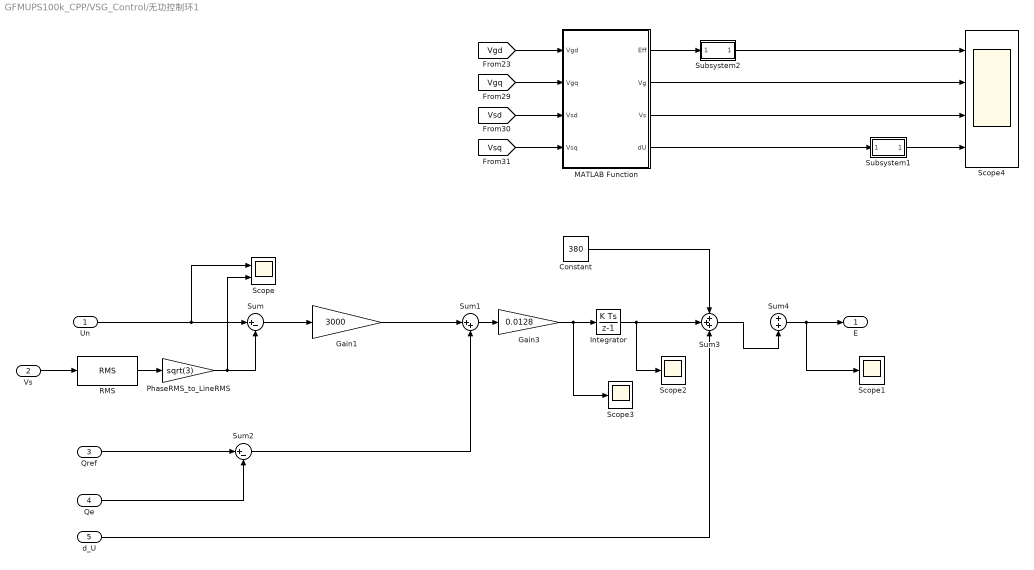
== system GFMUPS100k_CPP/VSG_Control/无功控制环1 ==
  Un : Inport
  Vs : Inport  Port=2
  Qref : Inport  Port=3
  Qe : Inport  Port=4
  d_U : Inport  Port=5
  Constant : Constant  Value=380  SampleTime=100e-6
  Gain1 : Gain  Gain=3000
  Gain3 : Gain  Gain=0.0128
  Integrator : DiscreteIntegrator  SampleTime=100e-6  ICPrevOutput=DiscIntNeverNeededParam  ICPrevScaledInput=DiscIntNeverNeededParam
  MATLAB Function : MATLAB Function  TreatAsAtomicUnit=on
  PhaseRMS_to_LineRMS : Gain  Gain=sqrt(3)
  RMS : dspstat3/RMS  run=off  directionMode=Each column  dimension=1  InputProcessing=Columns as channels (frame based)  reset_popup=None
  Scope : Scope  NumInputPorts=2
  Scope1 : Scope
  Scope2 : Scope
  Scope3 : Scope
  Scope4 : Scope  NumInputPorts=4
  Subsystem1 : Subsystem
  Subsystem2 : Subsystem
  Sum : Sum  Inputs=|+-
  Sum1 : Sum  Inputs=|++
  Sum2 : Sum  Inputs=|+-
  Sum3 : Sum  Inputs=+++
  Sum4 : Sum
  E : Outport
  wires:
  PhaseRMS_to_LineRMS/1 -> Scope/2, Sum/2
  RMS/1 -> PhaseRMS_to_LineRMS/1
  Sum2/1 -> Sum1/2
  Gain3/1 -> Scope3/1, Integrator/1
  Sum1/1 -> Gain3/1
  Un/1 -> Scope/1, Sum/1
  Qref/1 -> Sum2/1
  Sum/1 -> Gain1/1
  Vs/1 -> RMS/1
  Gain1/1 -> Sum1/1
  Qe/1 -> Sum2/2
  Constant/1 -> Sum3/1
  Integrator/1 -> Scope2/1, Sum3/2
  d_U/1 -> Sum3/3
  Sum3/1 -> Sum4/2
  Sum4/1 -> Scope1/1, E/1
  [Vgd] -> MATLAB Function/1(Vgd)
  [Vgq] -> MATLAB Function/2(Vgq)
  [Vsd] -> MATLAB Function/3(Vsd)
  [Vsq] -> MATLAB Function/4(Vsq)
  MATLAB Function/1(Eff) -> Subsystem2/1(In1)
  MATLAB Function/2(Vg) -> Scope4/2
  MATLAB Function/3(Vs) -> Scope4/3
  MATLAB Function/4(dU) -> Subsystem1/1(In1)
  Subsystem1/1(Out1) -> Scope4/4
  Subsystem2/1(Out1) -> Scope4/1

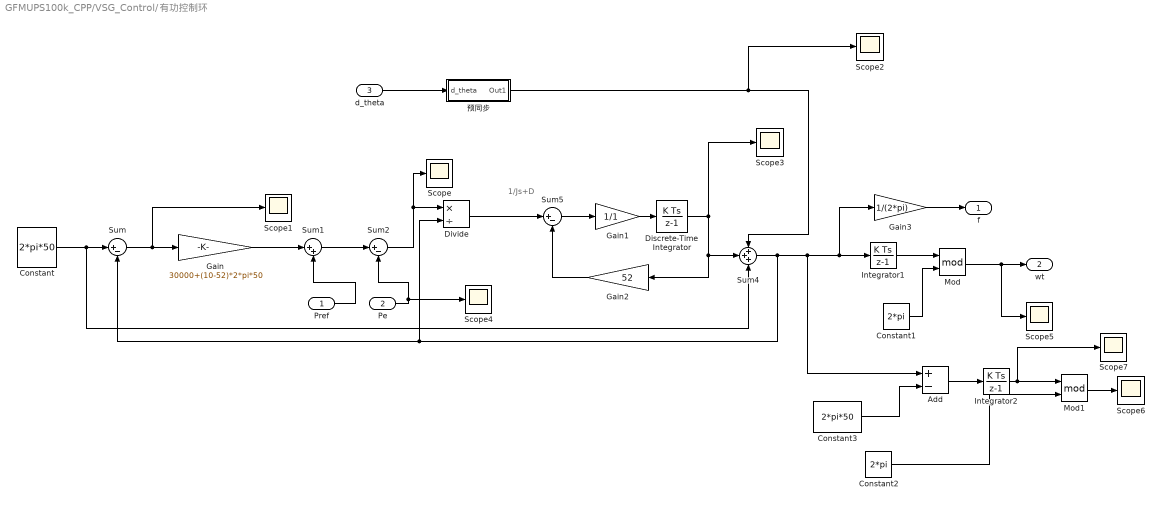
== system GFMUPS100k_CPP/VSG_Control/有功控制环 ==
  note: 1/Js+D
  Pref : Inport
  Pe : Inport  Port=2
  d_theta : Inport  Port=3
  Add : Sum  Inputs=+-
  Constant : Constant  Value=2*pi*50  SampleTime=100e-6
  Constant1 : Constant  Value=2*pi
  Constant2 : Constant  Value=2*pi
  Constant3 : Constant  Value=2*pi*50
  Discrete-Time Integrator : DiscreteIntegrator  SampleTime=5e-05  ICPrevOutput=DiscIntNeverNeededParam  ICPrevScaledInput=DiscIntNeverNeededParam
  Divide : Product  Inputs=*/
  Gain : Gain  Gain=30000+(10-52)*2*pi*50
  Gain1 : Gain  Gain=1/1
  Gain2 : Gain  Gain=52
  Gain3 : Gain  Gain=1/(2*pi)
  Integrator1 : DiscreteIntegrator  SampleTime=5e-05  ICPrevOutput=DiscIntNeverNeededParam  ICPrevScaledInput=DiscIntNeverNeededParam
  Integrator2 : DiscreteIntegrator  SampleTime=5e-05  ICPrevOutput=DiscIntNeverNeededParam  ICPrevScaledInput=DiscIntNeverNeededParam
  Mod : Math  Operator=mod
  Mod1 : Math  Operator=mod
  Scope{,1..7} (8 alike) : Scope
  Sum : Sum  Inputs=|+-
  Sum1 : Sum  Inputs=|++
  Sum2 : Sum  Inputs=|+-
  Sum4 : Sum  Inputs=+++
  Sum5 : Sum  Inputs=|+-
  预同步 : Subsystem
  f : Outport
  wt : Outport  Port=2
  wires:
  Sum/1 -> Gain/1, Scope1/1
  Gain/1 -> Sum1/1
  Constant/1 -> Sum4/3, Sum/1
  Sum2/1 -> Scope/1, Divide/1
  Mod/1 -> Scope5/1, wt/1
  Sum1/1 -> Sum2/1
  Integrator1/1 -> Mod/1
  Pe/1 -> Sum2/2, Scope4/1
  Gain3/1 -> f/1
  Constant1/1 -> Mod/2
  Discrete-Time Integrator/1 -> Sum4/2, Gain2/1, Scope3/1
  d_theta/1 -> 预同步/1(d_theta)
  预同步/1(Out1) -> Sum4/1, Scope2/1
  Sum5/1 -> Gain1/1
  Divide/1 -> Sum5/1
  Gain1/1 -> Discrete-Time Integrator/1
  Gain2/1 -> Sum5/2
  Pref/1 -> Sum1/2
  Constant2/1 -> Mod1/2
  Sum4/1 -> Divide/2, Sum/2, Add/1, Gain3/1, Integrator1/1
  Add/1 -> Integrator2/1
  Constant3/1 -> Add/2
  Mod1/1 -> Scope6/1
  Integrator2/1 -> Scope7/1, Mod1/1

== system GFMUPS100k_CPP/VSG_Control/虚拟阻抗（scr补偿） ==
  Ed : Inport
  Eq : Inport  Port=2
  id1 : Inport  Port=3
  iq1 : Inport  Port=4
  Gain : Gain  Gain=0.04398
  Gain1 : Gain  Gain=0.04398
  Gain2 : Gain  Gain=2*pi*50*1.4e-3
  Gain3 : Gain  Gain=2*pi*50*1.4e-3
  Subsystem1 : Subsystem
  Subsystem7 : Subsystem
  Sum1 : Sum  Inputs=|+-+
  Sum2 : Sum  Inputs=|+--
  Vdref1 : Outport
  Vqref1 : Outport  Port=2
  wires:
  Sum2/1 -> Vqref1/1
  Gain/1 -> Sum1/2
  Gain1/1 -> Sum2/2
  Gain2/1 -> Sum1/3
  Ed/1 -> Sum1/1
  Sum1/1 -> Vdref1/1
  Gain3/1 -> Sum2/3
  id1/1 -> Subsystem7/1(In1)
  iq1/1 -> Subsystem1/1(In1)
  Eq/1 -> Sum2/1
  Subsystem7/1(Out1) -> Gain/1, Gain3/1
  Subsystem1/1(Out1) -> Gain1/1, Gain2/1

== system GFMUPS100k_CPP/坐标变换1/Subsystem1 ==
  In1 : Inport
  Discrete-Time Integrator : DiscreteIntegrator  SampleTime=1/20000  ICPrevOutput=DiscIntNeverNeededParam  ICPrevScaledInput=DiscIntNeverNeededParam
  Gain1 : Gain  Gain=2*pi*20
  Gain2 : Gain
  Sum3 : Sum  Inputs=|+-
  Out1 : Outport
  wires:
  Sum3/1 -> Gain1/1
  Gain1/1 -> Discrete-Time Integrator/1
  Gain2/1 -> Sum3/2
  In1/1 -> Sum3/1
  Discrete-Time Integrator/1 -> Gain2/1, Out1/1

== system GFMUPS100k_CPP/坐标变换1/Subsystem2 ==
  In1 : Inport
  Discrete-Time Integrator : DiscreteIntegrator  SampleTime=1/20000  ICPrevOutput=DiscIntNeverNeededParam  ICPrevScaledInput=DiscIntNeverNeededParam
  Gain1 : Gain  Gain=2*pi*20
  Gain2 : Gain
  Sum3 : Sum  Inputs=|+-
  Out1 : Outport
  wires:
  Discrete-Time Integrator/1 -> Out1/1, Gain2/1
  In1/1 -> Sum3/1
  Gain2/1 -> Sum3/2
  Gain1/1 -> Discrete-Time Integrator/1
  Sum3/1 -> Gain1/1
